simulink model "s4"  (R2024b)
settings: Solver=FixedStepAuto  StartTime=0.0  StopTime=inf  RelTol=1e-3
InitFcn:
  | startSumoBridge
StartFcn:
  | addpath('D:\sim'); delete(findall(0,'Type','figure','Name','Simulink vs. SUMO Real-Time Response')); realtimeSumoMonitor();
StopFcn:
  | t_mon = timerfindall('Tag','SumoRealtimeMonitorTimer'); if ~isempty(t_mon), stop(t_mon); end
libraries: audiosources x1
settings Model: SimulationMode=accelerator  Creator=ma945  LastModifiedBy=ma945

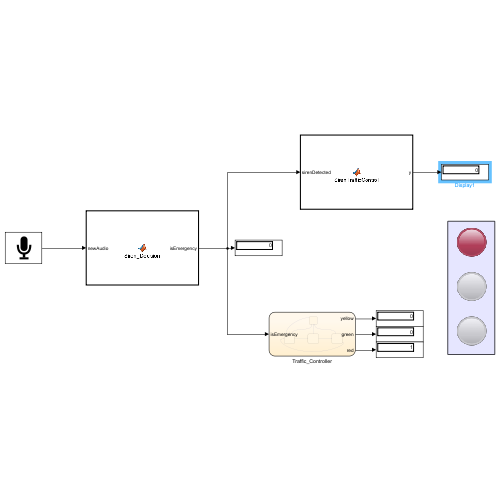
[thumbnail: Simulink's stored preview of the top-level diagram]
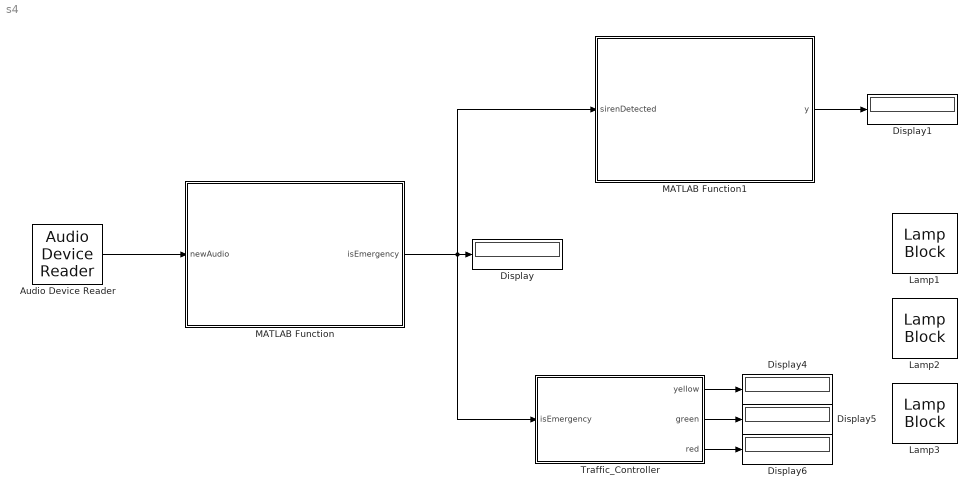
== system s4 ==
  Audio Device Reader : audiosources/Audio Device Reader  Driver=DirectSound  Device=Default  SampleRate=22050  NumChannels=1  SamplesPerFrame=11025  BitDepth=16-bit integer  NumBuffers=10  DefaultInputChannelMapping=on  InputChannelMapping=1:2  OutputNumOverrunSamples=off  OutputDataType=double  DriverIdx=1  DeviceWarnFlag=''
  Display{,1,4..6} (5 alike) : Display
  Lamp1 : LampBlock  LabelPosition=Hide
  Lamp2 : LampBlock  LabelPosition=Hide
  Lamp3 : LampBlock  LabelPosition=Hide
  MATLAB Function : MATLAB Function  TreatAsAtomicUnit=on
  MATLAB Function1 : MATLAB Function  TreatAsAtomicUnit=on
  Traffic_Controller : Stateflow chart  TreatAsAtomicUnit=on
  wires:
  Audio Device Reader/1 -> MATLAB Function/1(newAudio)
  Traffic_Controller/3(red) -> Display6/1
  Traffic_Controller/2(green) -> Display5/1
  Traffic_Controller/1(yellow) -> Display4/1
  MATLAB Function/1(isEmergency) -> MATLAB Function1/1(sirenDetected), Display/1, Traffic_Controller/1(isEmergency)
  MATLAB Function1/1(y) -> Display1/1

== matlab function s4/MATLAB Function1 ==
  data: sirenDetected input; y output

function y = SirenTrafficControl(sirenDetected)
%#codegen

coder.extrinsic('emergencyTrafficControl');

persistent lastState

if isempty(lastState)
    lastState = -1;
end

if sirenDetected >= 1
    currentState = 1;
else
    currentState = 0;
end

if currentState ~= lastState
    emergencyTrafficControl(currentState);
    lastState = currentState;
end

y = currentState;
end

== matlab function s4/MATLAB Function ==
  data: newAudio input; isEmergency output
function isEmergency = Siren_Decision(newAudio)
coder.extrinsic('detectSirenStep');

% تهيئة المخرج بنوع صريح
isEmergency = 0;
temp = 0;

% استدعاء الكشف مع تحويل النوع
temp = detectSirenStep(double(newAudio));
isEmergency = double(temp);
end

== stateflow chart s4/Traffic_Controller ==
  state entry_
    red = 0;
    yellow = 0;
    green = 1;
    note: isEmergency
  state entry_4
    red=1;
    yellow=0;
    green=0;
    note: red
  state entry_5
    red=0;
    yellow=1;
    green=0;
    note: yellow
  state entry_6
    red=0;
    yellow=0;
    green=1;
    note: green
  state95 -> state72 : after(10, sec) [isEmergency == 0]
  state72 -> state95 [order 2] : [isEmergency == 1]
  state78 -> state95 [order 2] : [isEmergency == 1]
  state75 -> state95 [order 2] : [isEmergency == 1]
  (default) -> state72
  state72 -> state78 [order 1] : after(20,sec) [isEmergency == 0]
  state75 -> state72 [order 1] : after(10,sec) [isEmergency == 0]
  state78 -> state75 [order 1] : after(2,sec) [isEmergency == 0]
  data: isEmergency input; yellow output; green output; red output
